simulink model "tb_rc_uart_line"  (R2026b)
values from neighbouring files (symbols this model uses):
  P = tc.P; P.rc.p_loss = 0    [t_rc_link.m]    (also in t_row_driver.m = shaddad_params('Assign', false); t_row_test_system.m = t_row_test_system.vcValue(res, 'P'))
  Ts = prm.Ts    [row_driver_bench.m]
settings Model: Creator=aomar  LastModifiedBy=aomar

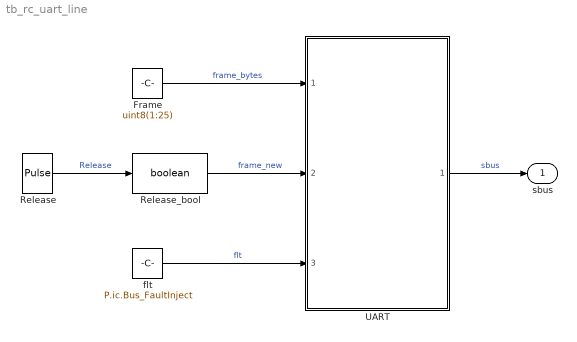
== system tb_rc_uart_line ==
  Frame : Constant  Value=uint8(1:25)  OutDataTypeStr=uint8  SampleTime=Ts.base
  Release : DiscretePulseGenerator  Period=round(P.rc.frame_period/Ts.base)  SampleTime=Ts.base
  Release_bool : DataTypeConversion  OutDataTypeStr=boolean  SaturateOnIntegerOverflow=off  RndMeth=Floor
  UART : Subsystem  ReferencedSubsystem=rc_uart_line_sim
  flt : Constant  Value=P.ic.Bus_FaultInject  OutDataTypeStr=Bus: Bus_FaultInject  SampleTime=Ts.base
  sbus : Outport  OutDataTypeStr=Bus: Bus_SbusStream
  wires:
  Release/1 -> Release_bool/1  "Release"
  Frame/1 -> UART/1  "frame_bytes"
  flt/1 -> UART/3  "flt"
  Release_bool/1 -> UART/2  "frame_new"
  UART/1 -> sbus/1  "sbus"
